simulink model "EFB_third_order"  (R2022b)
settings: Solver=FixedStepDiscrete  StartTime=0.0  StopTime=0.01  FixedStep=1e-8  RelTol=1e-3
libraries: dspsrcs4 x1
settings Model: Creator=ZIAD  LastModifiedBy=ASAA
settings OptimizationCC: ReuseModelBlockBuffer=on
settings RTWCC: GPUComputeCapability=5.0

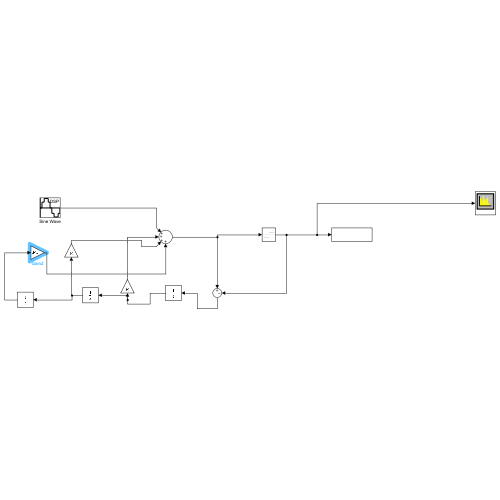
[thumbnail: Simulink's stored preview of the top-level diagram]
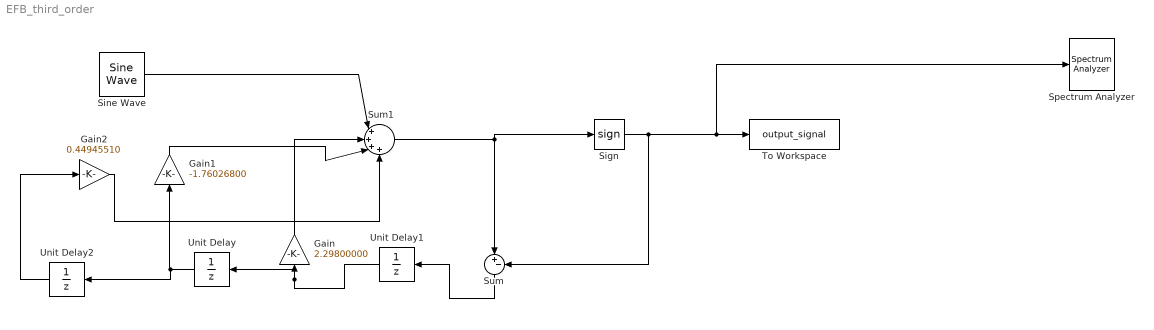
== system EFB_third_order ==
  Gain : Gain  Gain=2.29800000
  Gain1 : Gain  Gain=-1.76026800
  Gain2 : Gain  Gain=0.44945510
  Sign : Signum
  Sine Wave : dspsrcs4/Sine Wave  Amplitude=0.631  Frequency=100e3  Phase=0  SampleMode=Discrete  OutComplex=Real  CompMethod=Trigonometric fcn  TableSize=Speed  SampleTime=1/100e6  SamplesPerFrame=1  ResetState=Restart at time zero  OutputFrames=off  dataType=double  wordLen=16  udDataType=sfix(16)  fracBitsMode=Best precision  numFracBits=15  OutDataTypeStr=double  LastOutDataTypeStr=double
  Spectrum Analyzer : SpectrumAnalyzer
  Sum : Sum  Inputs=|+-
  Sum1 : Sum  Inputs=|++++
  To Workspace : ToWorkspace  VariableName=output_signal  SaveFormat=Timeseries  SampleTime=-1
  Unit Delay : UnitDelay  SampleTime=1e-8  HasFrameUpgradeWarning=on
  Unit Delay1 : UnitDelay  SampleTime=1e-8  HasFrameUpgradeWarning=on
  Unit Delay2 : UnitDelay  SampleTime=1e-8  HasFrameUpgradeWarning=on
  wires:
  Sum1/1 -> Sign/1, Sum/1
  Sign/1 -> Spectrum Analyzer/1, To Workspace/1, Sum/2
  Sum/1 -> Unit Delay1/1
  Sine Wave/1 -> Sum1/1
  Unit Delay1/1 -> Unit Delay/1, Gain/1
  Gain/1 -> Sum1/2
  Unit Delay/1 -> Gain1/1, Unit Delay2/1
  Unit Delay2/1 -> Gain2/1
  Gain1/1 -> Sum1/3
  Gain2/1 -> Sum1/4
